simulink model "sschdlexLVNLTransformerModel"  (R2026a)
settings: Solver=FixedStepDiscrete  StopTime=.2
libraries: fl_lib x18, ee_lib x6, nesl_utility x6
settings Model: DataTypeOverride=Off  Creator=The MathWorks, Inc.  LastModifiedBy=The MathWorks, Inc.
settings OptimizationCC: ConditionallyExecuteInputs=off  InheritOutputTypeSmallerThanSingle=on
settings DebuggingCC: ArtificialAlgebraicLoopMsg=error  SingleTaskRateTransMsg=error
settings HardwareCC: ProdHWDeviceType=ASIC/FPGA->ASIC/FPGA  TargetBitPerLong=64.0  TargetBitPerPointer=64.0  TargetBitPerSizeT=64.0  TargetBitPerPtrDiffT=64.0  TargetLongLongMode=on  TargetIntDivRoundTo=Zero  TargetEndianess=LittleEndian  TargetWordSize=64.0  TargetHWDeviceType=Custom Processor->MATLAB Host Computer  ProdEqTarget=off
settings SimscapeCC: SimscapeNominalValues="[{\"value\":\"1\",\"unit\":\"A\"},{\"value\":\"1\",\"unit\":\"bar\"},{\"value\":\"1\",\"unit\":\"cm^2\"},{\"value\":\"1\",\"unit\":\"cm^3/s\"},{\"value\":\"1\",\"unit\":\"kJ/kg\"},{\"value\":\"1\",\"unit\":\"kW\"},{\"value\":\"1\",\"unit\":\"l\"},{\"value\":\"1\",\"unit\":\"N\"},{\"value\":\"1\",\"unit\":\"N*m\"},{\"value\":\"1\",\"unit\":\"V\"}]"  SimscapeLogType=none  SimscapeLogDataHistory=5000.0

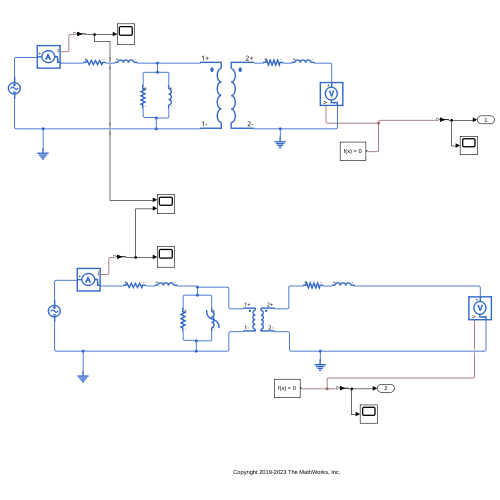
[thumbnail: Simulink's stored preview of the top-level diagram]
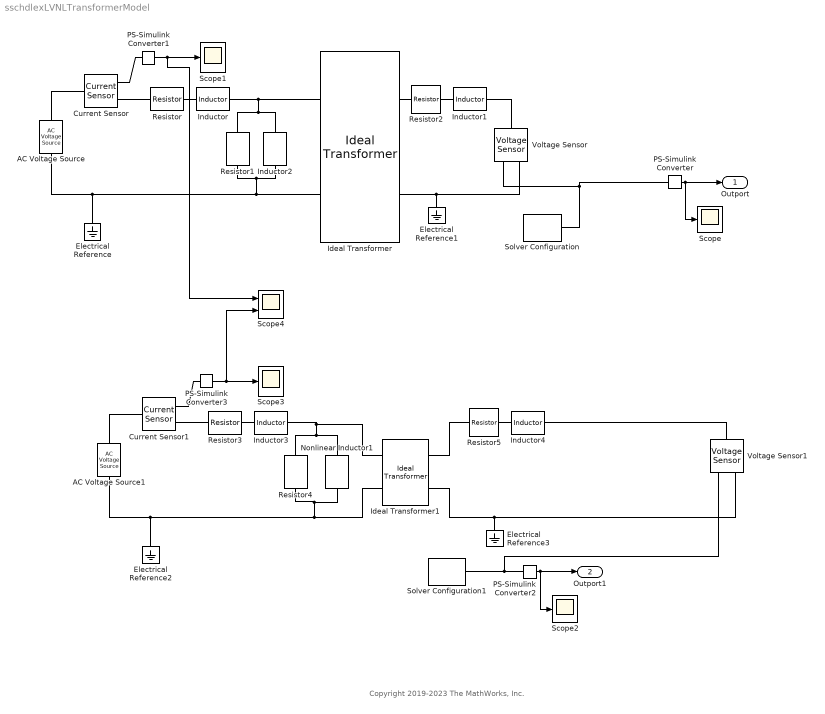
== system sschdlexLVNLTransformerModel ==
  note: Copyright 2019-2023 The MathWorks, Inc.
  AC Voltage Source : fl_lib/Electrical/Electrical Sources/AC Voltage Source  amp=328 V  shift=0 rad  frequency=60 Hz
  AC Voltage Source1 : fl_lib/Electrical/Electrical Sources/AC Voltage Source  amp=328 V  shift=0 rad  frequency=60 Hz
  Current Sensor : fl_lib/Electrical/Electrical Sensors/Current Sensor
  Current Sensor1 : fl_lib/Electrical/Electrical Sensors/Current Sensor
  Electrical Reference{,1..3} (4 alike) : fl_lib/Electrical/Electrical Elements/Electrical Reference
  Ideal Transformer : fl_lib/Electrical/Electrical Elements/Ideal Transformer  n=9.16666  i1_specify=off  i1_priority=None  i1=0 A  i1_nominal_specify=off  i1_nominal_value=1  i1_nominal_unit=A  v1_specify=off  v1_priority=None  v1=0 V  v1_nominal_specify=off  v1_nominal_value=1  v1_nominal_unit=V  i2_specify=off  i2_priority=None  i2=0 A  i2_nominal_specify=off  i2_nominal_value=1  i2_nominal_unit=A  v2_specify=off  v2_priority=None  v2=0 V  v2_nominal_specify=off  v2_nominal_value=1  v2_nominal_unit=V
  Ideal Transformer1 : fl_lib/Electrical/Electrical Elements/Ideal Transformer  n=9.16666  i1_specify=off  i1_priority=None  i1=0 A  i1_nominal_specify=off  i1_nominal_value=1  i1_nominal_unit=A  v1_specify=off  v1_priority=None  v1=0 V  v1_nominal_specify=off  v1_nominal_value=1  v1_nominal_unit=V  i2_specify=off  i2_priority=None  i2=0 A  i2_nominal_specify=off  i2_nominal_value=1  i2_nominal_unit=A  v2_specify=off  v2_priority=None  v2=0 V  v2_nominal_specify=off  v2_nominal_value=1  v2_nominal_unit=V
  Inductor : ee_lib/Passive/Inductor  l=2.54 mH  enable_L_tol=0  L_tol=20  tol_distribution=1  nSigma=4  r=0 Ohm  g=1e-9 1/Ohm  enable_operating_limits=0  operating_limit_action=2  max_working_current=1 A  power_rating=1 W  i_L_specify=off  i_L_priority=High  i_L=0 A  i_L_nominal_specify=off  i_L_nominal_value=1  i_L_nominal_unit=A
  Inductor1 : ee_lib/Passive/Inductor  l=2.54*9.1666 mH  enable_L_tol=0  L_tol=20  tol_distribution=1  nSigma=4  r=0 Ohm  g=1e-9 1/Ohm  enable_operating_limits=0  operating_limit_action=2  max_working_current=1 A  power_rating=1 W  i_L_specify=off  i_L_priority=High  i_L=0 A  i_L_nominal_specify=off  i_L_nominal_value=1  i_L_nominal_unit=A
  Inductor2 : ee_lib/Passive/Inductor  l=.75 H  enable_L_tol=0  L_tol=20  tol_distribution=1  nSigma=4  r=0 Ohm  g=1e-9 1/Ohm  enable_operating_limits=0  operating_limit_action=2  max_working_current=1 A  power_rating=1 W  i_L_specify=off  i_L_priority=High  i_L=0 A  i_L_nominal_specify=off  i_L_nominal_value=1  i_L_nominal_unit=A
  Inductor3 : ee_lib/Passive/Inductor  l=2.54 mH  enable_L_tol=0  L_tol=20  tol_distribution=1  nSigma=4  r=0 Ohm  g=1e-9 1/Ohm  enable_operating_limits=0  operating_limit_action=2  max_working_current=1 A  power_rating=1 W  i_L_specify=off  i_L_priority=High  i_L=0 A  i_L_nominal_specify=off  i_L_nominal_value=1  i_L_nominal_unit=A
  Inductor4 : ee_lib/Passive/Inductor  l=2.54*9.1666 mH  enable_L_tol=0  L_tol=20  tol_distribution=1  nSigma=4  r=0 Ohm  g=1e-9 1/Ohm  enable_operating_limits=0  operating_limit_action=2  max_working_current=1 A  power_rating=1 W  i_L_specify=off  i_L_priority=High  i_L=0 A  i_L_nominal_specify=off  i_L_nominal_value=1  i_L_nominal_unit=A
  Nonlinear Inductor1 : ee_lib/Passive/Nonlinear Inductor  parameterization_option=3  Nw=1  L=2e-4 H  L_sat=1e-4 H  current_data=[-8 -2 0 2 8] A  magnetic_flux_data=[-1.8 -1.5 0 1.5 1.8] Wb  H_data=[0, 200, 400, 600, 800, 1000] A/m  B_data=[0, .81, 1.25, 1.42, 1.48, 1.49] T  magnetic_flux_sat=1.3e-05 Wb  length_effective=0.032 m  area_effective=1.6e-5 m^2  dBdH0=0.005 m*T/A  B1=1.49 T  H1=1000 A/m  c=0.1  K=200 A/m  alpha=1e-4  averaging_period=0 s  G_parasitic=1e-9 1/Ohm  interpolation_option=1  x0_option=1  i_L0=0 A  phi0=0 Wb  B0=0 T  H0=0 A/m
  PS-Simulink Converter{,1..3} (4 alike) : nesl_utility/PS-Simulink Converter  PhysicalDomain=network_engine_domain  SubClassName=ps_output  LeftPortType=input  RightPortType=output  PseudoPeriodic=off  Frequencies=[]  VectorFormat=1-D array  Unit=1  AffineConversion=off
  Resistor : fl_lib/Electrical/Electrical Elements/Resistor  R=3.75 Ohm  i_specify=off  i_priority=None  i=0 A  i_nominal_specify=off  i_nominal_value=1  i_nominal_unit=A  v_specify=off  v_priority=None  v=0 V  v_nominal_specify=off  v_nominal_value=1  v_nominal_unit=V
  Resistor1 : fl_lib/Electrical/Electrical Elements/Resistor  R=3826 Ohm  i_specify=off  i_priority=None  i=0 A  i_nominal_specify=off  i_nominal_value=1  i_nominal_unit=A  v_specify=off  v_priority=None  v=0 V  v_nominal_specify=off  v_nominal_value=1  v_nominal_unit=V
  Resistor2 : fl_lib/Electrical/Electrical Elements/Resistor  R=3.75*9.1666 Ohm  i_specify=off  i_priority=None  i=0 A  i_nominal_specify=off  i_nominal_value=1  i_nominal_unit=A  v_specify=off  v_priority=None  v=0 V  v_nominal_specify=off  v_nominal_value=1  v_nominal_unit=V
  Resistor3 : fl_lib/Electrical/Electrical Elements/Resistor  R=3.75 Ohm  i_specify=off  i_priority=None  i=0 A  i_nominal_specify=off  i_nominal_value=1  i_nominal_unit=A  v_specify=off  v_priority=None  v=0 V  v_nominal_specify=off  v_nominal_value=1  v_nominal_unit=V
  Resistor4 : fl_lib/Electrical/Electrical Elements/Resistor  R=3826 Ohm  i_specify=off  i_priority=None  i=0 A  i_nominal_specify=off  i_nominal_value=1  i_nominal_unit=A  v_specify=off  v_priority=None  v=0 V  v_nominal_specify=off  v_nominal_value=1  v_nominal_unit=V
  Resistor5 : fl_lib/Electrical/Electrical Elements/Resistor  R=3.75*9.1666 Ohm  i_specify=off  i_priority=None  i=0 A  i_nominal_specify=off  i_nominal_value=1  i_nominal_unit=A  v_specify=off  v_priority=None  v=0 V  v_nominal_specify=off  v_nominal_value=1  v_nominal_unit=V
  Scope{,1..3} (4 alike) : Scope
      Scope settings: ActiveDisplayYMinimum=-45.00209  ActiveDisplayYMaximum=44.37507
      Scope1 settings: ActiveDisplayYMinimum=-1.92946  ActiveDisplayYMaximum=3.94455  DataLoggingSaveFormat=Array
      Scope2 settings: ActiveDisplayYMinimum=-44.86646  ActiveDisplayYMaximum=44.40549  DataLoggingVariableName=ScopeData2
      Scope3 settings: ActiveDisplayYMinimum=-1.92946  ActiveDisplayYMaximum=3.94455  DataLoggingVariableName=ScopeData3  DataLoggingSaveFormat=Array
  Scope4 : Scope  NumInputPorts=2
      settings: ActiveDisplayYMinimum=-1.53411  ActiveDisplayYMaximum=6.271  DataLoggingVariableName=ScopeData4
  Solver Configuration : nesl_utility/Solver Configuration  PhysicalDomain=network_engine_domain  SubClassName=solver  LeftPortType=input  RightPortType=generic  Tones=[]  Harmonics=[]  SimulateNoise=off  Profile=off  UseLocalSampling=off  EnableSwitchedLinearOptims=on  FrequencyDomain=off  UseCCode=off  RelTol=0.001  AbsTol=1e-06  MinStep=1e-09  ToWorkspace=off  RevertToSquareIcSolve=off  NumHomotopyIterations=100  PhasorMode=off  PhasorModeNumHarmonics=1  ConsistencySolver=NEWTON_FTOL  CanonicalOrdering=UNORDERED  OptimizeIntermediates=UNOPTIMIZED  IndexReductionMethod=DerivativeReplacement  DoDC=off  ResidualTolerance=1e-09  ConsistencyTolSource=GLOBAL  ConsistencyAbsTol=0.001  ConsistencyRelTol=0.001  ConsistencyTolFactor=0.001  UseLocalSolver=on  LocalSolverChoice=NE_PARTITIONING_ADVANCER  ResolveIndetEquations=on  FunctionEvalNumThread=1  LocalSolverSampleTime=1e-5  DoFixedCost=on  MaxNonlinIter=1  MaxModeIter=2  ComputeImpulses=off  ImpulseIterations=2  LinearAlgebra=auto  LinearAlgebraNumThread=0  EquationFormulation=NE_TIME_EF  DelaysMemoryBudget=1024  AutomaticFiltering=on  FilteringTimeConstant=0.001  PartitionStorageMethod=AS_NEEDED  PartitionMemoryBudget=1024  PartitionMethod=ROBUST  MultibodyUseLocalSolver=off  MultibodyLocalSolverChoice=ODE1  MultibodyLocalSolverSampleTime=0.001
  Solver Configuration1 : nesl_utility/Solver Configuration  PhysicalDomain=network_engine_domain  SubClassName=solver  LeftPortType=input  RightPortType=generic  Tones=[]  Harmonics=[]  SimulateNoise=off  Profile=off  UseLocalSampling=off  EnableSwitchedLinearOptims=on  FrequencyDomain=off  UseCCode=off  RelTol=0.001  AbsTol=1e-06  MinStep=1e-09  ToWorkspace=off  RevertToSquareIcSolve=off  NumHomotopyIterations=100  PhasorMode=off  PhasorModeNumHarmonics=1  ConsistencySolver=NEWTON_FTOL  CanonicalOrdering=UNORDERED  OptimizeIntermediates=UNOPTIMIZED  IndexReductionMethod=DerivativeReplacement  DoDC=off  ResidualTolerance=1e-09  ConsistencyTolSource=GLOBAL  ConsistencyAbsTol=0.001  ConsistencyRelTol=0.001  ConsistencyTolFactor=0.001  UseLocalSolver=on  LocalSolverChoice=NE_PARTITIONING_ADVANCER  ResolveIndetEquations=on  FunctionEvalNumThread=1  LocalSolverSampleTime=1e-5  DoFixedCost=on  MaxNonlinIter=1  MaxModeIter=2  ComputeImpulses=off  ImpulseIterations=2  LinearAlgebra=auto  LinearAlgebraNumThread=0  EquationFormulation=NE_TIME_EF  DelaysMemoryBudget=1024  AutomaticFiltering=on  FilteringTimeConstant=0.001  PartitionStorageMethod=AS_NEEDED  PartitionMemoryBudget=1024  PartitionMethod=ROBUST  MultibodyUseLocalSolver=off  MultibodyLocalSolverChoice=ODE1  MultibodyLocalSolverSampleTime=0.001
  Voltage Sensor : fl_lib/Electrical/Electrical Sensors/Voltage Sensor
  Voltage Sensor1 : fl_lib/Electrical/Electrical Sensors/Voltage Sensor
  Outport : Outport  VectorParamsAs1DForOutWhenUnconnected=off
  Outport1 : Outport  Port=2  VectorParamsAs1DForOutWhenUnconnected=off
  wires:
  PS-Simulink Converter/1 -> Scope/1, Outport/1
  PS-Simulink Converter3/1 -> Scope4/2, Scope3/1
  PS-Simulink Converter2/1 -> Scope2/1, Outport1/1
  PS-Simulink Converter1/1 -> Scope4/1, Scope1/1
  connections:
  Voltage Sensor/RConn1 -- PS-Simulink Converter/LConn1 -- Solver Configuration/RConn1
  Ideal Transformer/LConn2 -- Inductor2/RConn1 -- Resistor1/RConn1 -- AC Voltage Source/RConn1 -- Electrical Reference/LConn1
  Inductor/RConn1 -- Inductor2/LConn1 -- Resistor1/LConn1 -- Ideal Transformer/LConn1
  AC Voltage Source/LConn1 -- Current Sensor/LConn1
  Inductor/LConn1 -- Resistor/RConn1
  Current Sensor/RConn2 -- Resistor/LConn1
  Current Sensor/RConn1 -- PS-Simulink Converter1/LConn1
  Voltage Sensor/RConn2 -- Electrical Reference1/LConn1 -- Ideal Transformer/RConn2
  Ideal Transformer/RConn1 -- Resistor2/LConn1
  Inductor1/LConn1 -- Resistor2/RConn1
  Voltage Sensor/LConn1 -- Inductor1/RConn1
  Resistor4/RConn1 -- Nonlinear Inductor1/RConn1 -- Ideal Transformer1/LConn2 -- AC Voltage Source1/RConn1 -- Electrical Reference2/LConn1
  Electrical Reference3/LConn1 -- Voltage Sensor1/RConn2 -- Ideal Transformer1/RConn2
  Ideal Transformer1/LConn1 -- Nonlinear Inductor1/LConn1 -- Resistor4/LConn1 -- Inductor3/RConn1
  Voltage Sensor1/RConn1 -- PS-Simulink Converter2/LConn1 -- Solver Configuration1/RConn1
  AC Voltage Source1/LConn1 -- Current Sensor1/LConn1
  Inductor3/LConn1 -- Resistor3/RConn1
  Inductor4/LConn1 -- Resistor5/RConn1
  Current Sensor1/RConn2 -- Resistor3/LConn1
  Current Sensor1/RConn1 -- PS-Simulink Converter3/LConn1
  Ideal Transformer1/RConn1 -- Resistor5/LConn1
  Voltage Sensor1/LConn1 -- Inductor4/RConn1
